simulink model "scheme_L2_v9"  (R2026b)
settings: Solver=ode45  StopTime=10  MaxStep=0.005  RelTol=1e-9  AbsTol=1e-11
settings Model: Creator=Qndi  LastModifiedBy=Qndi

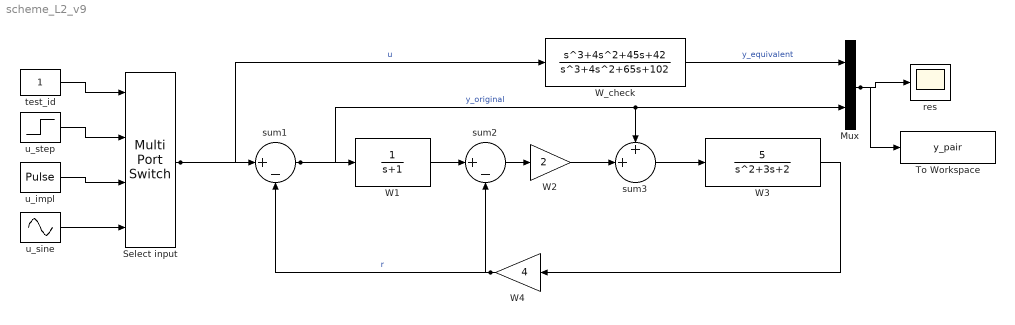
== system scheme_L2_v9 ==
  Mux : Mux  Inputs=2
  Select input : MultiPortSwitch  SaturateOnIntegerOverflow=off  InputSameDT=off
  To Workspace : ToWorkspace  VariableName=y_pair  SaveFormat=Timeseries  SampleTime=-1
  W1 : TransferFcn  Numerator=1  Denominator=[1 1]
  W2 : Gain  Gain=2
  W3 : TransferFcn  Numerator=5  Denominator=[1 3 2]
  W4 : Gain  Gain=4
  W_check : TransferFcn  Numerator=[1 4 45 42]  Denominator=[1 4 65 102]
  res : Scope
  sum1 : Sum  Inputs=|+-
  sum2 : Sum  Inputs=|+-
  sum3 : Sum  Inputs=++|
  test_id : Constant
  u_impl : DiscretePulseGenerator  PulseType=Time based  Amplitude=50  Period=20  PulseWidth=0.1  PhaseDelay=1
  u_sine : Sin  SampleTime=0
  u_step : Step  SampleTime=0
  wires:
  test_id/1 -> Select input/1
  u_step/1 -> Select input/2
  u_impl/1 -> Select input/3
  u_sine/1 -> Select input/4
  Select input/1 -> sum1/1, W_check/1  "u"
  sum1/1 -> W1/1, Mux/2, sum3/1  "y_original"
  W1/1 -> sum2/1
  sum2/1 -> W2/1
  W2/1 -> sum3/2
  sum3/1 -> W3/1
  W3/1 -> W4/1
  W4/1 -> sum1/2, sum2/2  "r"
  W_check/1 -> Mux/1  "y_equivalent"
  Mux/1 -> res/1, To Workspace/1
